simulink model "IEEE_BUS_68_AGC"  (R2025a)
settings: Solver=ode23tb  StartTime=0.0  StopTime=150  FixedStep=Ts  MaxStep=0.0001  RelTol=1e-3
PreLoadFcn:
  | PSSMODEL=1;
  | LPSS=0;
  | WAPSS=0;
  | WAPSS2=0;
  | Ts=50e-5;
InitFcn:
  | PSSMODEL=1;
  | LPSS=0;
  | WAPSS=0;
  | WAPSS2=0;
  | Ts=50e-5;
  | 
  | % Required data to 68 Bus benchmark
  | % clear
  | % clc
  | % Definition for the columns
  | % system base =100 MVA
  | 
  | %% Line data Format (line)
  | % All values are given on the same system base MVA
  | % 1: From bus
  | % 2: To bus
  | % 3: Resistance (pu)
  | % 4: Reactance  (pu)
  | % 5: Charge     (pu)
  | % 6: Transformer Tap Amplitute
  | % 7: base MVA
  | % 8: Nomonal Voltage (KV)
  | 
  | %1   2    3        4       5       6        7      8
  | line=[...
  | 1	54	0	     0.0181	  0	      1.025     100    13.8
  | 2	58	0	     0.025	  0	      1.070     100    13.8
  | 3	62	0	     0.02	  0	      1.070     100    13.8
  | 4	19	0.0007	 0.0142	  0	      1.070     100    13.8
  | 5	20	0.0009	 0.018	  0	      1.009     100    13.8
  | 6	22	0	     0.0143	  0	      1.025     100    13.8
  | 7	23	0.0005	 0.0272	  0	      0         100    13.8
  | 8	25	0.0006	 0.0232	  0	      1.025     100    13.8
  | 9	29	0.0008	 0.0156   0	      1.025     100    13.8
  | 10	31	0	     0.026	  0	      1.04      100    13.8
  | 11	32	0	     0.013	  0	      1.04      100    13.8
  | 12	36	0	     0.0075	  0	      1.04      100    13.8
  | 13	17	0	     0.0033	  0	      1.04      100    13.8
  | 14	41	0	     0.0015	  0	      1         100    13.8
  | 15	42	0	     0.0015	  0	      1         100    13.8
  | 16	18	0	     0.003	  0	      1         100    13.8
  | 17	36	0.0005	 0.0045	  0.32	  0         100    138
  | 17	43	0.0005	 0.0276	  0	      0         100    138
  | 18	42	0.004	 0.06	  2.25    0         100    138
  | 18	49	0.0076	 0.1141	  1.16    0	        100    138
  | 18	50	0.0012	 0.0288	  2.06	  0         100    138
  | 20	19	0.0007	 0.0138	  0       1.06	    100    138
  | 19	68	0.0016	 0.0195	  0.304	  0         100    138
  | 21	22	0.0008	 0.014	  0.2565  0	        100    138
  | 21	68	0.0008	 0.0135	  0.2548  0	        100    138
  | 22	23	0.0006	 0.0096	  0.1846  0	        100    138
  | 23	24	0.0022	 0.035	  0.361	  0         100    138
  | 24	68	0.0003	 0.0059	  0.068	  0         100    138
  | 25	26	0.0032	 0.0323	  0.531	  0         100    138
  | 25	54	0.007	 0.0086	  0.146	  0         100    138
  | 26	27	0.0014	 0.0147	  0.2396  0	        100    138
  | 26	28	0.0043	 0.0474	  0.7802  0	        100    138
  | 26	29	0.0057	 0.0625	  1.029	  0         100    138
  | 27	37	0.0013	 0.0173	  0.3216  0	        100    138
  | 27	53	0.032	 0.32	  0.41	  0         100    138
  | ... (+206 lines)
undefined symbols (not defined in the file or in its folder): D1, Delta
libraries: spsPMUPLLBasedPositiveSequenceLib x90, spsRMSLib x73, spsThreePhaseVIMeasurementLib x69, spsLoadFlowBusLib x69, spsThreePhasePISectionLineLib x64, spsThreePhaseParallelRLCLoadLib x35, spsGenericPowerSystemStabilizerLib x32, spsThreePhaseSeriesRLCLoadLib x21, spsThreePhaseTransformerTwoWindingsLib x21, spsSynchronousMachinepuStandardLib x20, spsExcitationSystemLib x16, spsMultiBandPowerSystemStabilizerLib x16
(part 2 of 8)

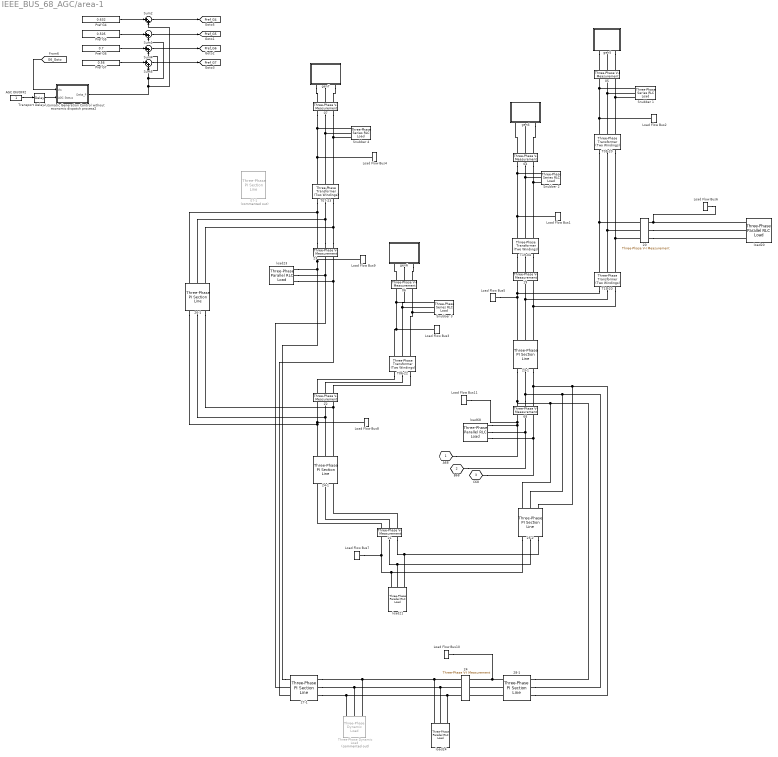
== system IEEE_BUS_68_AGC/area-1 ==
  04 : spsThreePhaseVIMeasurementLib/Three-Phase V-I Measurement  VoltageMeasurement=phase-to-phase  SetLabelV=on  LabelV=Vabc_04  Vpu=off  VpuLL=on  CurrentMeasurement=no  SetLabelI=off  LabelI=Iabc  Ipu=off  Pbase=100e6  Vbase=13.8*1e3  OutputType=Complex  PhasorSimulation=off  PSBequivalent=0
  05 : spsThreePhaseVIMeasurementLib/Three-Phase V-I Measurement  VoltageMeasurement=phase-to-phase  SetLabelV=on  LabelV=Vabc_05  Vpu=off  VpuLL=on  CurrentMeasurement=no  SetLabelI=off  LabelI=Iabc  Ipu=off  Pbase=100e6  Vbase=13.8e3  OutputType=Complex  PhasorSimulation=off  PSBequivalent=0
  06 : spsThreePhaseVIMeasurementLib/Three-Phase V-I Measurement  VoltageMeasurement=phase-to-phase  SetLabelV=on  LabelV=Vabc_06  Vpu=off  VpuLL=on  CurrentMeasurement=no  SetLabelI=off  LabelI=Iabc  Ipu=off  Pbase=100e6  Vbase=13.8e3  OutputType=Complex  PhasorSimulation=off  PSBequivalent=0
  07 : spsThreePhaseVIMeasurementLib/Three-Phase V-I Measurement  VoltageMeasurement=phase-to-phase  SetLabelV=on  LabelV=Vabc_07  Vpu=off  VpuLL=on  CurrentMeasurement=no  SetLabelI=off  LabelI=Iabc  Ipu=off  Pbase=100e6  Vbase=13.8e3  OutputType=Complex  PhasorSimulation=off  PSBequivalent=0
  07-1 : spsThreePhasePISectionLineLib/Three-Phase PI Section Line  Commented=on  LConnTagsString=a|b|c  RConnTagsString=A|B|C  Length=1  Frequency=60  Resistances=[line(7,3) 3*line(7,3)]  Inductances=[line(7,4) 3*line(7,4)]  Capacitances=[line(28,5) line(28,5)/3]
  19 : spsThreePhaseVIMeasurementLib/Three-Phase V-I Measurement  VoltageMeasurement=phase-to-phase  SetLabelV=on  LabelV=Vabc_19  Vpu=off  VpuLL=on  CurrentMeasurement=no  SetLabelI=off  LabelI=Iabc  Ipu=off  Pbase=100e6  Vbase=Bus(19,2)*1e3  OutputType=Complex  PhasorSimulation=off  PSBequivalent=0
  20 : spsThreePhaseVIMeasurementLib/Three-Phase V-I Measurement  VoltageMeasurement=phase-to-phase  SetLabelV=on  LabelV=Vabc_20  Vpu=off  VpuLL=on  CurrentMeasurement=no  SetLabelI=off  LabelI=Iabc  Ipu=off  Pbase=100e6  Vbase=Bus(20,2)*1e3  OutputType=Complex  PhasorSimulation=off  PSBequivalent=0
  21 : spsThreePhaseVIMeasurementLib/Three-Phase V-I Measurement  VoltageMeasurement=phase-to-phase  SetLabelV=on  LabelV=Vabc_21  Vpu=off  VpuLL=on  CurrentMeasurement=no  SetLabelI=off  LabelI=Iabc  Ipu=off  Pbase=100e6  Vbase=Bus(21,2)*1e3  OutputType=Complex  PhasorSimulation=off  PSBequivalent=0
  22 : spsThreePhaseVIMeasurementLib/Three-Phase V-I Measurement  VoltageMeasurement=phase-to-phase  SetLabelV=on  LabelV=Vabc_22  Vpu=off  VpuLL=on  CurrentMeasurement=no  SetLabelI=off  LabelI=Iabc  Ipu=off  Pbase=100e6  Vbase=Bus(22,2)*1e3  OutputType=Complex  PhasorSimulation=off  PSBequivalent=0
  23 : spsThreePhaseVIMeasurementLib/Three-Phase V-I Measurement  VoltageMeasurement=phase-to-phase  SetLabelV=on  LabelV=Vabc_23  Vpu=off  VpuLL=on  CurrentMeasurement=no  SetLabelI=off  LabelI=Iabc  Ipu=off  Pbase=100e6  Vbase=Bus(23,2)*1e3  OutputType=Complex  PhasorSimulation=off  PSBequivalent=0
  23-1 : spsThreePhasePISectionLineLib/Three-Phase PI Section Line  LConnTagsString=a|b|c  RConnTagsString=A|B|C  Length=1  Frequency=60  Resistances="[line(23,3)  3*line(23,3)]"  Inductances=[line(23,4) 3*line(23,4)]  Capacitances=[line(23,5) line(23,5)/3]
  24 : spsThreePhaseVIMeasurementLib/Three-Phase V-I Measurement  VoltageMeasurement=phase-to-phase  SetLabelV=on  LabelV=Vabc_24  Vpu=off  VpuLL=on  CurrentMeasurement=no  SetLabelI=off  LabelI=Iabc  Ipu=off  Pbase=100e6  Vbase=Bus(24,2)*1e3  OutputType=Complex  PhasorSimulation=off  PSBequivalent=0
  24-1 : spsThreePhasePISectionLineLib/Three-Phase PI Section Line  LConnTagsString=a|b|c  RConnTagsString=A|B|C  Length=1  Frequency=60  Resistances=[line(24,3) 3*line(24,3)]  Inductances=[line(24,4) 3*line(24,4)]  Capacitances=[line(24,5) line(24,5)/3]
  25-2 : spsThreePhasePISectionLineLib/Three-Phase PI Section Line  LConnTagsString=a|b|c  RConnTagsString=A|B|C  Length=1  Frequency=60  Resistances=[line(25,3) 3*line(25,3)]  Inductances=[line(25,4) 3*line(25,4)]  Capacitances=[line(25,5) line(25,5)/3]
  26-1 : spsThreePhasePISectionLineLib/Three-Phase PI Section Line  LConnTagsString=a|b|c  RConnTagsString=A|B|C  Length=1  Frequency=60  Resistances=[line(26,3) 3*line(26,3)]  Inductances=[line(26,4) 3*line(26,4)]  Capacitances=[line(26,5) line(26,5)/3]
  27-1 : spsThreePhasePISectionLineLib/Three-Phase PI Section Line  LConnTagsString=a|b|c  RConnTagsString=A|B|C  Length=1  Frequency=60  Resistances=[line(27,3) 3*line(27,3)]  Inductances=[line(27,4) 3*line(27,4)]  Capacitances=[line(27,5) line(27,5)/3]
  28-1 : spsThreePhasePISectionLineLib/Three-Phase PI Section Line  LConnTagsString=a|b|c  RConnTagsString=A|B|C  Length=1  Frequency=60  Resistances=[line(28,3) 3*line(28,3)]  Inductances=[line(28,4) 3*line(28,4)]  Capacitances=[line(28,5) line(28,5)/3]
  68 : spsThreePhaseVIMeasurementLib/Three-Phase V-I Measurement  VoltageMeasurement=phase-to-phase  SetLabelV=on  LabelV=Vabc_68  Vpu=off  VpuLL=on  CurrentMeasurement=no  SetLabelI=off  LabelI=Iabc  Ipu=off  Pbase=100e6  Vbase=Bus(68,2)*1e3  OutputType=Complex  PhasorSimulation=off  PSBequivalent=0
  AGC ON/OFF2 : Constant
  Automatic Generation Control without economic dispatch process2 : Subsystem
  Load Flow Bus1 : spsLoadFlowBusLib/Load Flow Bus  LConnTagsString=a  Phases=single  Connectors=on one side  ID=BUS_04  Vbase=13.8e3  Vref=0.997  Vangle=0  VLF=0.997  VLFb=1  VLFc=1  angleLF=-1.084  angleLFb=0  angleLFc=0
  Load Flow Bus10 : spsLoadFlowBusLib/Load Flow Bus  LConnTagsString=a  Phases=single  Connectors=on one side  ID=BUS_24  Vbase=138e3  Vref=1  Vangle=0  VLF=1.017  VLFb=1  VLFc=1  angleLF=18.89  angleLFb=0  angleLFc=0
  Load Flow Bus11 : spsLoadFlowBusLib/Load Flow Bus  LConnTagsString=a  Phases=single  Connectors=on one side  ID=BUS_68  Vbase=138e3  Vref=1  Vangle=0  VLF=1.009  VLFb=1  VLFc=1  angleLF=18.71  angleLFb=0  angleLFc=0
  Load Flow Bus2 : spsLoadFlowBusLib/Load Flow Bus  LConnTagsString=a  Phases=single  Connectors=on one side  ID=BUS_05  Vbase=13.8e3  Vref=1.011  Vangle=0  VLF=1.011  VLFb=1  VLFc=1  angleLF=-5.107  angleLFb=0  angleLFc=0
  Load Flow Bus3 : spsLoadFlowBusLib/Load Flow Bus  LConnTagsString=a  Phases=single  Connectors=on one side  ID=BUS_06  Vbase=13.8e3  Vref=1.05  Vangle=0  VLF=1.05  VLFb=1  VLFc=1  angleLF=-1.181  angleLFb=0  angleLFc=0
  Load Flow Bus4 : spsLoadFlowBusLib/Load Flow Bus  LConnTagsString=a  Phases=single  Connectors=on one side  ID=BUS_07  Vbase=13.8e3  Vref=1.063  Vangle=0  VLF=1.063  VLFb=1  VLFc=1  angleLF=-0.2085  angleLFb=0  angleLFc=0
  Load Flow Bus5 : spsLoadFlowBusLib/Load Flow Bus  LConnTagsString=a  Phases=single  Connectors=on one side  ID=BUS_19  Vbase=138e3  Vref=1  Vangle=0  VLF=0.9998  VLFb=1  VLFc=1  angleLF=23.76  angleLFb=0  angleLFc=0
  Load Flow Bus6 : spsLoadFlowBusLib/Load Flow Bus  LConnTagsString=a  Phases=single  Connectors=on one side  ID=BUS_20  Vbase=138e3  Vref=1  Vangle=0  VLF=0.9971  VLFb=1  VLFc=1  angleLF=22.34  angleLFb=0  angleLFc=0
  Load Flow Bus7 : spsLoadFlowBusLib/Load Flow Bus  LConnTagsString=a  Phases=single  Connectors=on one side  ID=BUS_21  Vbase=138e3  Vref=1  Vangle=0  VLF=1.014  VLFb=1  VLFc=1  angleLF=21.41  angleLFb=0  angleLFc=0
  Load Flow Bus8 : spsLoadFlowBusLib/Load Flow Bus  LConnTagsString=a  Phases=single  Connectors=on one side  ID=BUS_22  Vbase=138e3  Vref=1  Vangle=0  VLF=1.039  VLFb=1  VLFc=1  angleLF=26.18  angleLFb=0  angleLFc=0
  Load Flow Bus9 : spsLoadFlowBusLib/Load Flow Bus  LConnTagsString=a  Phases=single  Connectors=on one side  ID=BUS_23  Vbase=138e3  Vref=1  Vangle=0  VLF=1.039  VLFb=1  VLFc=1  angleLF=25.85  angleLFb=0  angleLFc=0
  Pref G4 : Constant  Value=0.632
  Pref G5 : Constant  Value=0.505
  Pref G6 : Constant  Value=0.7
  Pref G7 : Constant  Value=0.56
  Snubber {1..4} (4 alike) : spsThreePhaseSeriesRLCLoadLib/Three-Phase Series RLC Load  LConnTagsString=A|B|C  Configuration=Y (grounded)  NominalVoltage=13.8e3  Vabc=[1e3 1e3 1e3]  Vabcp=[1e3 1e3 1e3]  NominalFrequency=60  UnbalancedPower=off  ActivePower=1000000  InductivePower=0  CapacitivePower=10000000  Pabc=[10e3 9e3 11e3]  QLabc=[100 90 110]  QCabc=[100 90 110]  Pabcp=[10e3 9e3 11e3]  QLabcp=[100 90 110]  QCabcp=[100 90 110]  Measurements=None  LoadType=constant Z
  Sum{1..2,4..5} (4 alike) : Sum  Inputs=|++
  T05-20 : spsThreePhaseTransformerTwoWindingsLib/Three-Phase Transformer (Two Windings)  Winding1Connection=Delta (D1)  Winding2Connection=Yg  CoreType=Three single-phase transformers  SetSaturation=off  Hysteresis=off  DataFile='hysteresis'  SetInitialFlux=off  Measurements=None  UNITS=pu  NominalPower=[ 100e6 , 60 ]  Winding1=[ 13.8e3 , 0.0, 0 ]  Winding2=[ 138e3 , 0.00085, 0.0091]  Rm=500  Lm=500  L0=0.5  Saturation=[ 0,0 ; 0.0024,1.2 ; 1.0,1.52 ]  InitialFluxes=[ 0.8 , -0.8 , 0.7 ]  BreakLoop=off  DiscreteSolver=Trapezoidal robust  DataType=off  TransfoNumber=1
  T06-22 : spsThreePhaseTransformerTwoWindingsLib/Three-Phase Transformer (Two Windings)  Winding1Connection=Delta (D1)  Winding2Connection=Yg  CoreType=Three single-phase transformers  SetSaturation=off  Hysteresis=off  DataFile='hysteresis'  SetInitialFlux=off  Measurements=None  UNITS=pu  NominalPower=[ 100e6 , 60 ]  Winding1=[ 13.8e3 , 0.00 , 0 ]  Winding2=[ 138e3 , 0.000 , 0.0072 ]  Rm=500  Lm=500  L0=0.5  Saturation=[ 0,0 ; 0.0024,1.2 ; 1.0,1.52 ]  InitialFluxes=[ 0.8 , -0.8 , 0.7 ]  BreakLoop=off  DiscreteSolver=Trapezoidal robust  DataType=off  TransfoNumber=1
  T07-23 : spsThreePhaseTransformerTwoWindingsLib/Three-Phase Transformer (Two Windings)  Winding1Connection=Delta (D1)  Winding2Connection=Yg  CoreType=Three single-phase transformers  SetSaturation=off  Hysteresis=off  DataFile='hysteresis'  SetInitialFlux=off  Measurements=None  UNITS=pu  NominalPower=[ 100e6 , 60 ]  Winding1=[ 13.8e3 , 0.00035 , 0 ]  Winding2=[ 138e3 , 0.00035, 0.0138]  Rm=500  Lm=500  L0=0.5  Saturation=[ 0,0 ; 0.0024,1.2 ; 1.0,1.52 ]  InitialFluxes=[ 0.8 , -0.8 , 0.7 ]  BreakLoop=off  DiscreteSolver=Trapezoidal robust  DataType=off  TransfoNumber=1
  T19-04 : spsThreePhaseTransformerTwoWindingsLib/Three-Phase Transformer (Two Windings)  Winding1Connection=Delta (D1)  Winding2Connection=Yg  CoreType=Three single-phase transformers  SetSaturation=off  Hysteresis=off  DataFile='hysteresis'  SetInitialFlux=off  Measurements=None  UNITS=pu  NominalPower=[ 100e6 , 60 ]  Winding1=[ 13.8e3 , 0.00035 , 0 ]  Winding2=[ 138e3 , 0.000035, 0.0142]  Rm=500  Lm=500  L0=0.5  Saturation=[ 0,0 ; 0.0024,1.2 ; 1.0,1.52 ]  InitialFluxes=[ 0.8 , -0.8 , 0.7 ]  BreakLoop=off  DiscreteSolver=Trapezoidal robust  DataType=off  TransfoNumber=1
  T19-20 : spsThreePhaseTransformerTwoWindingsLib/Three-Phase Transformer (Two Windings)  Winding1Connection=Y  Winding2Connection=Y  CoreType=Three single-phase transformers  SetSaturation=off  Hysteresis=off  DataFile='hysteresis'  SetInitialFlux=off  Measurements=None  UNITS=pu  NominalPower=[ 100e6 , 60 ]  Winding1=[ 138e3 , 0.00035 , 0 ]  Winding2=[ 138e3 , 0.00035, 0.0138]  Rm=500  Lm=500  L0=0.5  Saturation=[ 0,0 ; 0.0024,1.2 ; 1.0,1.52 ]  InitialFluxes=[ 0.8 , -0.8 , 0.7 ]  BreakLoop=off  DiscreteSolver=Trapezoidal robust  DataType=off  TransfoNumber=1
  Three-Phase Dynamic Load : spsThreePhaseDynamicLoadLib/Three-Phase Dynamic Load  Commented=on  NominalVoltage=[138000 60 ]  ActiveReactivePowers=[309000000 -92000000]  PositiveSequence=[1.01116 21.5615]  ExternalControl=off  NpNq=[1.3 2]  TimeConstants=[0.1 0.1 0.1 0.1]  MinimumVoltage=0.5  Tfilter=0.01  LoadFlowParameters=[4,0,0,0,0]
      settings: LibrarySourceBlock=|
      | sps_lib/Passives/Three-Phase
      | Dynamic Load
  Transport Delay2 : TransportDelay  DelayTime=20
  gen4 : Subsystem
  gen5 : Subsystem
  gen6 : Subsystem
  gen7 : Subsystem
  load20 : spsThreePhaseParallelRLCLoadLib/Three-Phase Parallel RLC Load  LConnTagsString=A|B|C  Configuration=Y (grounded)  NominalVoltage=(138000)*0.997073  Vabc=[1e3 1e3 1e3]  Vabcp=[1e3 1e3 1e3]  NominalFrequency=60  UnbalancedPower=off  ActivePower=680000000  InductivePower=103000000  CapacitivePower=0  Pabc=[10e3 9e3 11e3]  QLabc=[100 90 110]  QCabc=[100 90 110]  Pabcp=[10e3 9e3 11e3]  QLabcp=[100 90 110]  QCabcp=[100 90 110]  Measurements=None  LoadType=constant PQ
  load21 : spsThreePhaseParallelRLCLoadLib/Three-Phase Parallel RLC Load  LConnTagsString=A|B|C  Configuration=Y (grounded)  NominalVoltage=(138000)*1.01427  Vabc=[1e3 1e3 1e3]  Vabcp=[1e3 1e3 1e3]  NominalFrequency=60  UnbalancedPower=off  ActivePower=274000000  InductivePower=115000000  CapacitivePower=0  Pabc=[10e3 9e3 11e3]  QLabc=[100 90 110]  QCabc=[100 90 110]  Pabcp=[10e3 9e3 11e3]  QLabcp=[100 90 110]  QCabcp=[100 90 110]  Measurements=None  LoadType=constant PQ
  load23 : spsThreePhaseParallelRLCLoadLib/Three-Phase Parallel RLC Load  LConnTagsString=A|B|C  Configuration=Y (grounded)  NominalVoltage=(138000)*1.03943  Vabc=[1e3 1e3 1e3]  Vabcp=[1e3 1e3 1e3]  NominalFrequency=60  UnbalancedPower=off  ActivePower=248000000  InductivePower=85000000  CapacitivePower=0  Pabc=[10e3 9e3 11e3]  QLabc=[100 90 110]  QCabc=[100 90 110]  Pabcp=[10e3 9e3 11e3]  QLabcp=[100 90 110]  QCabcp=[100 90 110]  Measurements=None  LoadType=constant PQ
  load24 : spsThreePhaseParallelRLCLoadLib/Three-Phase Parallel RLC Load  LConnTagsString=A|B|C  Configuration=Y (grounded)  NominalVoltage=(138000)*1.01674  Vabc=[1e3 1e3 1e3]  Vabcp=[1e3 1e3 1e3]  NominalFrequency=60  UnbalancedPower=off  ActivePower=309000000  InductivePower=0  CapacitivePower=92000000  Pabc=[10e3 9e3 11e3]  QLabc=[100 90 110]  QCabc=[100 90 110]  Pabcp=[10e3 9e3 11e3]  QLabcp=[100 90 110]  QCabcp=[100 90 110]  Measurements=None  LoadType=constant PQ
  load68 : spsThreePhaseParallelRLCLoadLib/Three-Phase Parallel RLC Load  LConnTagsString=A|B|C  Configuration=Y (grounded)  NominalVoltage=(138000)*1.00875  Vabc=[1e3 1e3 1e3]  Vabcp=[1e3 1e3 1e3]  NominalFrequency=60  UnbalancedPower=off  ActivePower=329000000  InductivePower=32000000  CapacitivePower=0  Pabc=[10e3 9e3 11e3]  QLabc=[100 90 110]  QCabc=[100 90 110]  Pabcp=[10e3 9e3 11e3]  QLabcp=[100 90 110]  QCabcp=[100 90 110]  Measurements=None  LoadType=constant PQ
  A68 : PMIOPort  Tag=PMCPort  Side=Right
  B68 : PMIOPort  Tag=PMCPort  Port=2  Side=Right
  C68 : PMIOPort  Tag=PMCPort  Port=3  Side=Right
  tag scope: Pref_G4=global, Pref_G5=global, Pref_G6=global, Pref_G7=global
  wires:
  Sum2/1 -> [Pref_G4]
  Sum1/1 -> [Pref_G5]
  Pref G6/1 -> Sum4/1
  Sum5/1 -> [Pref_G7]
  Automatic Generation Control without economic dispatch process2/1(Delta_P) -> Sum2/2, Sum1/2, Sum4/2, Sum5/2
  Pref G4/1 -> Sum2/1
  Sum4/1 -> [Pref_G6]
  Pref G5/1 -> Sum1/1
  Pref G7/1 -> Sum5/1
  [G6_Goto] -> Automatic Generation Control without economic dispatch process2/1(dw)
  AGC ON/OFF2/1 -> Transport Delay2/1
  Transport Delay2/1 -> Automatic Generation Control without economic dispatch process2/2(AGC Status)
  ? -> ?
  ? -> ?
  ? -> ?
  ? -> ?
  connections:
  B68/RConn1 -- load68/LConn2 -- 68/LConn2
  27-1/LConn1 -- Load Flow Bus9/LConn1 -- 23/LConn1 -- load23/LConn1
  T19-20/LConn3 -- T05-20/RConn3 -- 20/RConn3
  20/RConn1 -- T05-20/RConn1 -- T19-20/LConn1
  24-1/RConn1 -- 26-1/RConn1 -- Load Flow Bus8/LConn1 -- 22/LConn1
  04/LConn2 -- T19-04/LConn2 -- Snubber 2/LConn2
  07/LConn1 -- Snubber 4/LConn1 -- Load Flow Bus4/LConn1 -- T07-23/LConn1
  07/LConn3 -- T07-23/LConn3 -- Snubber 4/LConn3
  load23/LConn2 -- 23/LConn2 -- 27-1/LConn2
  21/LConn3 -- load21/LConn3 -- 25-2/RConn3
  24-1/RConn3 -- 22/LConn3 -- 26-1/RConn3
  04/LConn1 -- Snubber 2/LConn1 -- Load Flow Bus1/LConn1 -- T19-04/LConn1
  A68/RConn1 -- load68/LConn1 -- 68/LConn1 -- Load Flow Bus11/LConn1
  04/RConn1 -- gen4/LConn1
  T19-20/LConn2 -- T05-20/RConn2 -- 20/RConn2
  23-1/RConn1 -- Load Flow Bus5/LConn1 -- T19-20/RConn1 -- 19/LConn1
  21/LConn2 -- load21/LConn2 -- 25-2/RConn2
  load23/LConn3 -- 23/LConn3 -- 27-1/LConn3
  T06-22/RConn3 -- 22/RConn3
  07/LConn2 -- Snubber 4/LConn2 -- T07-23/LConn2
  load21/LConn1 -- Load Flow Bus7/LConn1 -- 21/LConn1 -- 25-2/RConn1
  C68/RConn1 -- load68/LConn3 -- 68/LConn3
  T06-22/LConn1 -- Load Flow Bus3/LConn1 -- Snubber 3/LConn1 -- 06/LConn1
  T05-20/LConn1 -- Load Flow Bus2/LConn1 -- Snubber 1/LConn1 -- 05/LConn1
  T06-22/LConn3 -- 06/LConn3 -- Snubber 3/LConn3
  26-1/RConn2 -- 24-1/RConn2 -- 22/LConn2
  T06-22/LConn2 -- Snubber 3/LConn2 -- 06/LConn2
  04/LConn3 -- Snubber 2/LConn3 -- T19-04/LConn3
  T06-22/RConn2 -- 22/RConn2
  gen4/LConn2 -- 04/RConn2
  23-1/LConn1 -- 68/RConn1 -- 28-1/LConn1 -- 25-2/LConn1
  T19-04/RConn3 -- 19/RConn3
  68/RConn2 -- 23-1/LConn2 -- 28-1/LConn2 -- 25-2/LConn2
  T06-22/RConn1 -- 22/RConn1
  T19-04/RConn2 -- 19/RConn2
  28-1/LConn3 -- 68/RConn3 -- 23-1/LConn3 -- 25-2/LConn3
  gen4/LConn3 -- 04/RConn3
  19/LConn2 -- 23-1/RConn2 -- T19-20/RConn2
  T19-04/RConn1 -- 19/RConn1
  T05-20/LConn2 -- Snubber 1/LConn2 -- 05/LConn2
  T05-20/LConn3 -- Snubber 1/LConn3 -- 05/LConn3
  gen5/LConn1 -- 05/RConn1
  gen5/LConn2 -- 05/RConn2
  gen5/LConn3 -- 05/RConn3
  06/RConn1 -- gen6/LConn1
  gen6/LConn2 -- 06/RConn2
  gen6/LConn3 -- 06/RConn3
  gen7/LConn1 -- 07/RConn1
  gen7/LConn2 -- 07/RConn2
  gen7/LConn3 -- 07/RConn3
  19/LConn3 -- 23-1/RConn3 -- T19-20/RConn3
  23/RConn1 -- T07-23/RConn1 -- 26-1/LConn1
  23/RConn2 -- T07-23/RConn2 -- 26-1/LConn2
  23/RConn3 -- T07-23/RConn3 -- 26-1/LConn3
  21/RConn1 -- 24-1/LConn1
  21/RConn2 -- 24-1/LConn2
  21/RConn3 -- 24-1/LConn3
  28-1/RConn1 -- 24/LConn1 -- Load Flow Bus10/LConn1
  28-1/RConn2 -- 24/LConn2
  28-1/RConn3 -- 24/LConn3
  Load Flow Bus6/LConn1 -- load20/LConn1 -- 20/LConn1
  27-1/RConn1 -- load24/LConn1 -- 24/RConn1 -- Three-Phase Dynamic Load/LConn1
  24/RConn2 -- Three-Phase Dynamic Load/LConn2 -- 27-1/RConn2 -- load24/LConn2
  24/RConn3 -- Three-Phase Dynamic Load/LConn3 -- 27-1/RConn3 -- load24/LConn3
  20/LConn2 -- load20/LConn2
  20/LConn3 -- load20/LConn3

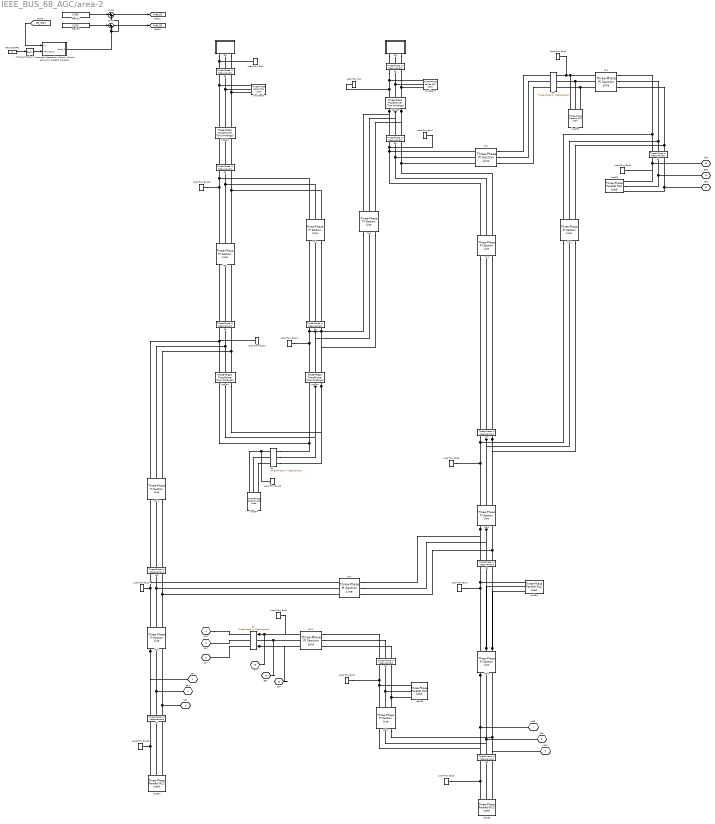
== system IEEE_BUS_68_AGC/area-2 ==
  02 : spsThreePhaseVIMeasurementLib/Three-Phase V-I Measurement  VoltageMeasurement=phase-to-phase  SetLabelV=on  LabelV=Vabc_02  Vpu=off  VpuLL=on  CurrentMeasurement=no  SetLabelI=off  LabelI=Iabc  Ipu=off  Pbase=100e6  Vbase=13.8e3  OutputType=Complex  PhasorSimulation=off  PSBequivalent=0
  03 : spsThreePhaseVIMeasurementLib/Three-Phase V-I Measurement  VoltageMeasurement=phase-to-phase  SetLabelV=on  LabelV=Vabc_03  Vpu=off  VpuLL=on  CurrentMeasurement=no  SetLabelI=off  LabelI=Iabc  Ipu=off  Pbase=100e6  Vbase=13.8e3  OutputType=Complex  PhasorSimulation=off  PSBequivalent=0
  37 : spsThreePhaseVIMeasurementLib/Three-Phase V-I Measurement  VoltageMeasurement=phase-to-phase  SetLabelV=on  LabelV=Vabc_37  Vpu=off  VpuLL=on  CurrentMeasurement=no  SetLabelI=off  LabelI=Iabc  Ipu=off  Pbase=100e6  Vbase=Bus(37,2)*1e3  OutputType=Complex  PhasorSimulation=off  PSBequivalent=0
  50-1 : spsThreePhasePISectionLineLib/Three-Phase PI Section Line  LConnTagsString=a|b|c  RConnTagsString=A|B|C  Length=1  Frequency=60  Resistances=[line(50,3) 3*line(50,3)]  Inductances=[line(50,4) 3*line(50,4)]  Capacitances=[line(50,5) line(50,5)/3]
  52 : spsThreePhaseVIMeasurementLib/Three-Phase V-I Measurement  VoltageMeasurement=phase-to-phase  SetLabelV=on  LabelV=Vabc_52  Vpu=off  VpuLL=on  CurrentMeasurement=no  SetLabelI=off  LabelI=Iabc  Ipu=off  Pbase=100e6  Vbase=Bus(52,2)*1e3  OutputType=Complex  PhasorSimulation=off  PSBequivalent=0
  55 : spsThreePhaseVIMeasurementLib/Three-Phase V-I Measurement  VoltageMeasurement=phase-to-phase  SetLabelV=on  LabelV=Vabc_55  Vpu=off  VpuLL=on  CurrentMeasurement=no  SetLabelI=off  LabelI=Iabc  Ipu=off  Pbase=100e6  Vbase=Bus(55,2)*1e3  OutputType=Complex  PhasorSimulation=off  PSBequivalent=0
  56 : spsThreePhaseVIMeasurementLib/Three-Phase V-I Measurement  VoltageMeasurement=phase-to-phase  SetLabelV=on  LabelV=Vabc_56  Vpu=off  VpuLL=on  CurrentMeasurement=no  SetLabelI=off  LabelI=Iabc  Ipu=off  Pbase=100e6  Vbase=Bus(56,2)*1e3  OutputType=Complex  PhasorSimulation=off  PSBequivalent=0
  57 : spsThreePhaseVIMeasurementLib/Three-Phase V-I Measurement  VoltageMeasurement=phase-to-phase  SetLabelV=on  LabelV=Vabc_57  Vpu=off  VpuLL=on  CurrentMeasurement=no  SetLabelI=off  LabelI=Iabc  Ipu=off  Pbase=100e6  Vbase=Bus(57,2)*1e3  OutputType=Complex  PhasorSimulation=off  PSBequivalent=0
  58 : spsThreePhaseVIMeasurementLib/Three-Phase V-I Measurement  VoltageMeasurement=phase-to-phase  SetLabelV=on  LabelV=Vabc_58  Vpu=off  VpuLL=on  CurrentMeasurement=no  SetLabelI=off  LabelI=Iabc  Ipu=off  Pbase=100e6  Vbase=Bus(58,2)*1e3  OutputType=Complex  PhasorSimulation=off  PSBequivalent=0
  59 : spsThreePhaseVIMeasurementLib/Three-Phase V-I Measurement  VoltageMeasurement=phase-to-phase  SetLabelV=on  LabelV=Vabc_59  Vpu=off  VpuLL=on  CurrentMeasurement=no  SetLabelI=off  LabelI=Iabc  Ipu=off  Pbase=100e6  Vbase=Bus(59,2)*1e3  OutputType=Complex  PhasorSimulation=off  PSBequivalent=0
  60 : spsThreePhaseVIMeasurementLib/Three-Phase V-I Measurement  VoltageMeasurement=phase-to-phase  SetLabelV=on  LabelV=Vabc_60  Vpu=off  VpuLL=on  CurrentMeasurement=no  SetLabelI=off  LabelI=Iabc  Ipu=off  Pbase=100e6  Vbase=Bus(60,2)*1e3  OutputType=Complex  PhasorSimulation=off  PSBequivalent=0
  62 : spsThreePhaseVIMeasurementLib/Three-Phase V-I Measurement  VoltageMeasurement=phase-to-phase  SetLabelV=on  LabelV=Vabc_62  Vpu=off  VpuLL=on  CurrentMeasurement=no  SetLabelI=off  LabelI=Iabc  Ipu=off  Pbase=100e6  Vbase=Bus(62,2)*1e3  OutputType=Complex  PhasorSimulation=off  PSBequivalent=0
  63 : spsThreePhaseVIMeasurementLib/Three-Phase V-I Measurement  VoltageMeasurement=phase-to-phase  SetLabelV=on  LabelV=Vabc_63  Vpu=off  VpuLL=on  CurrentMeasurement=no  SetLabelI=off  LabelI=Iabc  Ipu=off  Pbase=100e6  Vbase=Bus(63,2)*1e3  OutputType=Complex  PhasorSimulation=off  PSBequivalent=0
  64 : spsThreePhaseVIMeasurementLib/Three-Phase V-I Measurement  VoltageMeasurement=phase-to-phase  SetLabelV=on  LabelV=Vabc_64  Vpu=off  VpuLL=on  CurrentMeasurement=no  SetLabelI=off  LabelI=Iabc  Ipu=off  Pbase=100e6  Vbase=Bus(64,2)*1e3  OutputType=Complex  PhasorSimulation=off  PSBequivalent=0
  65 : spsThreePhaseVIMeasurementLib/Three-Phase V-I Measurement  VoltageMeasurement=phase-to-phase  SetLabelV=on  LabelV=Vabc_65  Vpu=off  VpuLL=on  CurrentMeasurement=no  SetLabelI=off  LabelI=Iabc  Ipu=off  Pbase=100e6  Vbase=Bus(65,2)*1e3  OutputType=Complex  PhasorSimulation=off  PSBequivalent=0
  65-1 : spsThreePhasePISectionLineLib/Three-Phase PI Section Line  LConnTagsString=a|b|c  RConnTagsString=A|B|C  Length=1  Frequency=60  Resistances=[line(65,3) 3*line(65,3)]  Inductances=[line(65,4) 3*line(65,4)]  Capacitances=[line(65,5) line(65,5)/3]
  66 : spsThreePhaseVIMeasurementLib/Three-Phase V-I Measurement  VoltageMeasurement=phase-to-phase  SetLabelV=on  LabelV=Vabc_66  Vpu=off  VpuLL=on  CurrentMeasurement=no  SetLabelI=off  LabelI=Iabc  Ipu=off  Pbase=100e6  Vbase=Bus(66,2)*1e3  OutputType=Complex  PhasorSimulation=off  PSBequivalent=0
  67 : spsThreePhaseVIMeasurementLib/Three-Phase V-I Measurement  VoltageMeasurement=phase-to-phase  SetLabelV=on  LabelV=Vabc_67  Vpu=off  VpuLL=on  CurrentMeasurement=no  SetLabelI=off  LabelI=Iabc  Ipu=off  Pbase=100e6  Vbase=Bus(67,2)*1e3  OutputType=Complex  PhasorSimulation=off  PSBequivalent=0
  68-1 : spsThreePhasePISectionLineLib/Three-Phase PI Section Line  LConnTagsString=a|b|c  RConnTagsString=A|B|C  Length=1  Frequency=60  Resistances=[line(68,3) 3*line(68,3)]  Inductances=[line(68,4) 3*line(68,4)]  Capacitances=[line(68,5) line(68,5)/3]
  69-1 : spsThreePhasePISectionLineLib/Three-Phase PI Section Line  LConnTagsString=a|b|c  RConnTagsString=A|B|C  Length=1  Frequency=60  Resistances=[line(69,3) 3*line(69,3)]  Inductances=[line(69,4) 3*line(69,4)]  Capacitances=[line(69,5) line(69,5)/3]
  70-1 : spsThreePhasePISectionLineLib/Three-Phase PI Section Line  LConnTagsString=a|b|c  RConnTagsString=A|B|C  Length=1  Frequency=60  Resistances=[line(70,3) 3*line(70,3)]  Inductances=[line(70,4) 3*line(70,4)]  Capacitances=[line(70,5) line(70,5)/3]
  71-1 : spsThreePhasePISectionLineLib/Three-Phase PI Section Line  LConnTagsString=a|b|c  RConnTagsString=A|B|C  Length=1  Frequency=60  Resistances=[line(71,3) 3*line(71,3)]  Inductances=[line(71,4) 3*line(71,4)]  Capacitances=[line(71,5) line(71,5)/3]
  72-1 : spsThreePhasePISectionLineLib/Three-Phase PI Section Line  LConnTagsString=a|b|c  RConnTagsString=A|B|C  Length=1  Frequency=60  Resistances=[line(72,3) 3*line(72,3)]  Inductances=[line(72,4) 3*line(72,4)]  Capacitances=[line(72,5) line(72,5)/3]
  73-1 : spsThreePhasePISectionLineLib/Three-Phase PI Section Line  LConnTagsString=a|b|c  RConnTagsString=A|B|C  Length=1  Frequency=60  Resistances=[line(73,3) 3*line(73,3)]  Inductances=[line(73,4) 3*line(73,4)]  Capacitances=[line(73,5) line(73,5)/3]
  74-1 : spsThreePhasePISectionLineLib/Three-Phase PI Section Line  LConnTagsString=a|b|c  RConnTagsString=A|B|C  Length=1  Frequency=60  Resistances=[line(74,3) 3*line(74,3)]  Inductances=[line(74,4) 3*line(74,4)]  Capacitances=[line(74,5) line(74,5)/3]
  75-1 : spsThreePhasePISectionLineLib/Three-Phase PI Section Line  LConnTagsString=a|b|c  RConnTagsString=A|B|C  Length=1  Frequency=60  Resistances=[line(75,3) 3*line(75,3)]  Inductances=[line(75,4) 3*line(75,4)]  Capacitances=[line(75,5) line(75,5)/3]
  77-1 : spsThreePhasePISectionLineLib/Three-Phase PI Section Line  LConnTagsString=a|b|c  RConnTagsString=A|B|C  Length=1  Frequency=60  Resistances=[line(77,3) 3*line(77,3)]  Inductances=[line(77,4) 3*line(77,4)]  Capacitances=[line(77,5) line(77,5)/3]
  78-1 : spsThreePhasePISectionLineLib/Three-Phase PI Section Line  LConnTagsString=a|b|c  RConnTagsString=A|B|C  Length=1  Frequency=60  Resistances=[line(78,3) 3*line(78,3)]  Inductances=[line(78,4) 3*line(78,4)]  Capacitances=[line(78,5) line(78,5)/3]
  81-1 : spsThreePhasePISectionLineLib/Three-Phase PI Section Line  LConnTagsString=a|b|c  RConnTagsString=A|B|C  Length=1  Frequency=60  Resistances=[line(81,3) 3*line(81,3)]  Inductances=[line(81,4) 3*line(81,4)]  Capacitances=[line(81,5) line(81,5)/3]
  81-2 : spsThreePhasePISectionLineLib/Three-Phase PI Section Line  LConnTagsString=a|b|c  RConnTagsString=A|B|C  Length=1  Frequency=60  Resistances=[line(81,3) 3*line(81,3)]  Inductances=[line(81,4) 3*line(81,4)]  Capacitances=[line(81,5) line(81,5)/3]
  AGC ON/OFF2 : Constant
  Automatic Generation Control without economic dispatch process2 : Subsystem
  G2 : Subsystem
  G3 : Subsystem
  Load Flow Bus : spsLoadFlowBusLib/Load Flow Bus  LConnTagsString=a  Phases=single  Connectors=on one side  ID=BUS_02  Vbase=13.8e3  Vref=0.98  Vangle=0  VLF=0.98  VLFb=1  VLFc=1  angleLF=-12.66  angleLFb=0  angleLFc=0
  Load Flow Bus1 : spsLoadFlowBusLib/Load Flow Bus  LConnTagsString=a  Phases=single  Connectors=on one side  ID=BUS_03  Vbase=13.8e3  Vref=0.983  Vangle=0  VLF=0.983  VLFb=1  VLFc=1  angleLF=-5.973  angleLFb=0  angleLFc=0
  Load Flow Bus10 : spsLoadFlowBusLib/Load Flow Bus  LConnTagsString=a  Phases=single  Connectors=on one side  ID=BUS_62  Vbase=138e3  Vref=1  Vangle=0  VLF=0.9822  VLFb=1  VLFc=1  angleLF=20.14  angleLFb=0  angleLFc=0
  Load Flow Bus11 : spsLoadFlowBusLib/Load Flow Bus  LConnTagsString=a  Phases=single  Connectors=on one side  ID=BUS_63  Vbase=138e3  Vref=1  Vangle=0  VLF=0.9798  VLFb=1  VLFc=1  angleLF=19.17  angleLFb=0  angleLFc=0
  Load Flow Bus12 : spsLoadFlowBusLib/Load Flow Bus  LConnTagsString=a  Phases=single  Connectors=on one side  ID=BUS_64  Vbase=138e3  Vref=1  Vangle=0  VLF=0.9711  VLFb=1  VLFc=1  angleLF=19.33  angleLFb=0  angleLFc=0
  Load Flow Bus13 : spsLoadFlowBusLib/Load Flow Bus  LConnTagsString=a  Phases=single  Connectors=on one side  ID=BUS_65  Vbase=138e3  Vref=1  Vangle=0  VLF=0.9826  VLFb=1  VLFc=1  angleLF=19.44  angleLFb=0  angleLFc=0
  Load Flow Bus14 : spsLoadFlowBusLib/Load Flow Bus  LConnTagsString=a  Phases=single  Connectors=on one side  ID=BUS_66  Vbase=138e3  Vref=1  Vangle=0  VLF=0.988  VLFb=1  VLFc=1  angleLF=17.89  angleLFb=0  angleLFc=0
  Load Flow Bus15 : spsLoadFlowBusLib/Load Flow Bus  LConnTagsString=a  Phases=single  Connectors=on one side  ID=BUS_67  Vbase=138e3  Vref=1  Vangle=0  VLF=0.9976  VLFb=1  VLFc=1  angleLF=17.99  angleLFb=0  angleLFc=0
  Load Flow Bus2 : spsLoadFlowBusLib/Load Flow Bus  LConnTagsString=a  Phases=single  Connectors=on one side  ID=BUS_52  Vbase=138e3  Vref=1  Vangle=0  VLF=1.005  VLFb=1  VLFc=1  angleLF=15.5  angleLFb=0  angleLFc=0
  Load Flow Bus3 : spsLoadFlowBusLib/Load Flow Bus  LConnTagsString=a  Phases=single  Connectors=on one side  ID=BUS_55  Vbase=138e3  Vref=1  Vangle=0  VLF=0.9931  VLFb=1  VLFc=1  angleLF=13.46  angleLFb=0  angleLFc=0
  Load Flow Bus4 : spsLoadFlowBusLib/Load Flow Bus  LConnTagsString=a  Phases=single  Connectors=on one side  ID=BUS_56  Vbase=138e3  Vref=1  Vangle=0  VLF=0.9815  VLFb=1  VLFc=1  angleLF=15.77  angleLFb=0  angleLFc=0
  Load Flow Bus5 : spsLoadFlowBusLib/Load Flow Bus  LConnTagsString=a  Phases=single  Connectors=on one side  ID=BUS_37  Vbase=138e3  Vref=1  Vangle=0  VLF=1.011  VLFb=1  VLFc=1  angleLF=16.75  angleLFb=0  angleLFc=0
  Load Flow Bus6 : spsLoadFlowBusLib/Load Flow Bus  LConnTagsString=a  Phases=single  Connectors=on one side  ID=BUS_57  Vbase=138e3  Vref=1  Vangle=0  VLF=0.9777  VLFb=1  VLFc=1  angleLF=16.56  angleLFb=0  angleLFc=0
  Load Flow Bus7 : spsLoadFlowBusLib/Load Flow Bus  LConnTagsString=a  Phases=single  Connectors=on one side  ID=BUS_58  Vbase=138e3  Vref=1  Vangle=0  VLF=0.9787  VLFb=1  VLFc=1  angleLF=17.29  angleLFb=0  angleLFc=0
  Load Flow Bus8 : spsLoadFlowBusLib/Load Flow Bus  LConnTagsString=a  Phases=single  Connectors=on one side  ID=BUS_59  Vbase=138e3  Vref=1  Vangle=0  VLF=0.9696  VLFb=1  VLFc=1  angleLF=14.76  angleLFb=0  angleLFc=0
  Load Flow Bus9 : spsLoadFlowBusLib/Load Flow Bus  LConnTagsString=a  Phases=single  Connectors=on one side  ID=BUS_60  Vbase=138e3  Vref=1  Vangle=0  VLF=0.9697  VLFb=1  VLFc=1  angleLF=14.12  angleLFb=0  angleLFc=0
  Pref G2 : Constant  Value=0.545
  Pref G3 : Constant  Value=0.325
  Snubber 8 : spsThreePhaseSeriesRLCLoadLib/Three-Phase Series RLC Load  LConnTagsString=A|B|C  Configuration=Y (grounded)  NominalVoltage=13.8e3  Vabc=[1e3 1e3 1e3]  Vabcp=[1e3 1e3 1e3]  NominalFrequency=60  UnbalancedPower=off  ActivePower=1000000  InductivePower=0  CapacitivePower=10000000  Pabc=[10e3 9e3 11e3]  QLabc=[100 90 110]  QCabc=[100 90 110]  Pabcp=[10e3 9e3 11e3]  QLabcp=[100 90 110]  QCabcp=[100 90 110]  Measurements=None  LoadType=constant Z
  Snubber 9 : spsThreePhaseSeriesRLCLoadLib/Three-Phase Series RLC Load  LConnTagsString=A|B|C  Configuration=Y (grounded)  NominalVoltage=13.8e3  Vabc=[1e3 1e3 1e3]  Vabcp=[1e3 1e3 1e3]  NominalFrequency=60  UnbalancedPower=off  ActivePower=1000000  InductivePower=0  CapacitivePower=10000000  Pabc=[10e3 9e3 11e3]  QLabc=[100 90 110]  QCabc=[100 90 110]  Pabcp=[10e3 9e3 11e3]  QLabcp=[100 90 110]  QCabcp=[100 90 110]  Measurements=None  LoadType=constant Z
  Sum4 : Sum  Inputs=|++
  Sum5 : Sum  Inputs=|++
  T02-58 : spsThreePhaseTransformerTwoWindingsLib/Three-Phase Transformer (Two Windings)  Winding1Connection=Delta (D1)  Winding2Connection=Yg  CoreType=Three single-phase transformers  SetSaturation=off  Hysteresis=off  DataFile='hysteresis'  SetInitialFlux=off  Measurements=None  UNITS=pu  NominalPower=[ 100e6 , 60 ]  Winding1=[ 13.8e3 , 0.0002 , 0 ]  Winding2=[ 138e3 , 0 .0002, 0.0125]  Rm=500  Lm=500  L0=0.5  Saturation=[ 0,0 ; 0.0024,1.2 ; 1.0,1.52 ]  InitialFluxes=[ 0.8 , -0.8 , 0.7 ]  BreakLoop=off  DiscreteSolver=Trapezoidal robust  DataType=off  TransfoNumber=1
  T03-62 : spsThreePhaseTransformerTwoWindingsLib/Three-Phase Transformer (Two Windings)  Winding1Connection=Delta (D1)  Winding2Connection=Yg  CoreType=Three single-phase transformers  SetSaturation=off  Hysteresis=off  DataFile='hysteresis'  SetInitialFlux=off  Measurements=None  UNITS=pu  NominalPower=[ 100e6 , 60 ]  Winding1=[ 13.8e3 , 0.000 , 0 ]  Winding2=[ 138e3 , 0.000, 0.0101]  Rm=500  Lm=500  L0=0.5  Saturation=[ 0,0 ; 0.0024,1.2 ; 1.0,1.52 ]  InitialFluxes=[ 0.8 , -0.8 , 0.7 ]  BreakLoop=off  DiscreteSolver=Trapezoidal robust  DataType=off  TransfoNumber=1
  T63-64 : spsThreePhaseTransformerTwoWindingsLib/Three-Phase Transformer (Two Windings)  Winding1Connection=Y  Winding2Connection=Y  CoreType=Three single-phase transformers  SetSaturation=off  Hysteresis=off  DataFile='hysteresis'  SetInitialFlux=off  Measurements=None  UNITS=pu  NominalPower=[ 100e6 , 60 ]  Winding1=[ 138e3 , 0.00152, 0 ]  Winding2=[ 138e3 , 0.00152 , 0.022]  Rm=500  Lm=500  L0=0.5  Saturation=[ 0,0 ; 0.0024,1.2 ; 1.0,1.52 ]  InitialFluxes=[ 0.8 , -0.8 , 0.7 ]  BreakLoop=off  DiscreteSolver=Trapezoidal robust  DataType=off  TransfoNumber=1
  T65-64 : spsThreePhaseTransformerTwoWindingsLib/Three-Phase Transformer (Two Windings)  Winding1Connection=Y  Winding2Connection=Y  CoreType=Three single-phase transformers  SetSaturation=off  Hysteresis=off  DataFile='hysteresis'  SetInitialFlux=off  Measurements=None  UNITS=pu  NominalPower=[ 100e6 , 60 ]  Winding1=[ 138e3 , 0.00152, 0 ]  Winding2=[ 138e3 , 0.00152 , 0.022]  Rm=500  Lm=500  L0=0.5  Saturation=[ 0,0 ; 0.0024,1.2 ; 1.0,1.52 ]  InitialFluxes=[ 0.8 , -0.8 , 0.7 ]  BreakLoop=off  DiscreteSolver=Trapezoidal robust  DataType=off  TransfoNumber=1
  Transport Delay2 : TransportDelay  DelayTime=20
  load52 : spsThreePhaseParallelRLCLoadLib/Three-Phase Parallel RLC Load  LConnTagsString=A|B|C  Configuration=Y (grounded)  NominalVoltage=(138000)*1.00456  Vabc=[1e3 1e3 1e3]  Vabcp=[1e3 1e3 1e3]  NominalFrequency=60  UnbalancedPower=off  ActivePower=2000000  InductivePower=460000  CapacitivePower=0  Pabc=[10e3 9e3 11e3]  QLabc=[100 90 110]  QCabc=[100 90 110]  Pabcp=[10e3 9e3 11e3]  QLabcp=[100 90 110]  QCabcp=[100 90 110]  Measurements=None  LoadType=constant PQ
  load55 : spsThreePhaseParallelRLCLoadLib/Three-Phase Parallel RLC Load  LConnTagsString=A|B|C  Configuration=Y (grounded)  NominalVoltage=(138000)*0.993139  Vabc=[1e3 1e3 1e3]  Vabcp=[1e3 1e3 1e3]  NominalFrequency=60  UnbalancedPower=off  ActivePower=680000000  InductivePower=157000000  CapacitivePower=0  Pabc=[10e3 9e3 11e3]  QLabc=[100 90 110]  QCabc=[100 90 110]  Pabcp=[10e3 9e3 11e3]  QLabcp=[100 90 110]  QCabcp=[100 90 110]  Measurements=None  LoadType=constant PQ
  load56 : spsThreePhaseParallelRLCLoadLib/Three-Phase Parallel RLC Load  LConnTagsString=A|B|C  Configuration=Y (grounded)  NominalVoltage=(138000)*0.981548  Vabc=[1e3 1e3 1e3]  Vabcp=[1e3 1e3 1e3]  NominalFrequency=60  UnbalancedPower=off  ActivePower=200000000  InductivePower=74000000  CapacitivePower=0  Pabc=[10e3 9e3 11e3]  QLabc=[100 90 110]  QCabc=[100 90 110]  Pabcp=[10e3 9e3 11e3]  QLabcp=[100 90 110]  QCabcp=[100 90 110]  Measurements=None  LoadType=constant PQ
  load59 : spsThreePhaseParallelRLCLoadLib/Three-Phase Parallel RLC Load  LConnTagsString=A|B|C  Configuration=Y (grounded)  NominalVoltage=(138000)*0.969624  Vabc=[1e3 1e3 1e3]  Vabcp=[1e3 1e3 1e3]  NominalFrequency=60  UnbalancedPower=off  ActivePower=234000000  InductivePower=84000000  CapacitivePower=0  Pabc=[10e3 9e3 11e3]  QLabc=[100 90 110]  QCabc=[100 90 110]  Pabcp=[10e3 9e3 11e3]  QLabcp=[100 90 110]  QCabcp=[100 90 110]  Measurements=None  LoadType=constant PQ
  load60 : spsThreePhaseParallelRLCLoadLib/Three-Phase Parallel RLC Load  LConnTagsString=A|B|C  Configuration=Y (grounded)  NominalVoltage=(138000)*0.969673  Vabc=[1e3 1e3 1e3]  Vabcp=[1e3 1e3 1e3]  NominalFrequency=60  UnbalancedPower=off  ActivePower=209000000  InductivePower=71000000  CapacitivePower=0  Pabc=[10e3 9e3 11e3]  QLabc=[100 90 110]  QCabc=[100 90 110]  Pabcp=[10e3 9e3 11e3]  QLabcp=[100 90 110]  QCabcp=[100 90 110]  Measurements=None  LoadType=constant PQ
  load64 : spsThreePhaseParallelRLCLoadLib/Three-Phase Parallel RLC Load  LConnTagsString=A|B|C  Configuration=Y (grounded)  NominalVoltage=(138000)*0.971077  Vabc=[1e3 1e3 1e3]  Vabcp=[1e3 1e3 1e3]  NominalFrequency=60  UnbalancedPower=off  ActivePower=9000000  InductivePower=88000000  CapacitivePower=0  Pabc=[10e3 9e3 11e3]  QLabc=[100 90 110]  QCabc=[100 90 110]  Pabcp=[10e3 9e3 11e3]  QLabcp=[100 90 110]  QCabcp=[100 90 110]  Measurements=None  LoadType=constant PQ
  load67 : spsThreePhaseParallelRLCLoadLib/Three-Phase Parallel RLC Load  LConnTagsString=A|B|C  Configuration=Y (grounded)  NominalVoltage=(138000)*0.997643  Vabc=[1e3 1e3 1e3]  Vabcp=[1e3 1e3 1e3]  NominalFrequency=60  UnbalancedPower=off  ActivePower=118000000  InductivePower=27000000  CapacitivePower=0  Pabc=[10e3 9e3 11e3]  QLabc=[100 90 110]  QCabc=[100 90 110]  Pabcp=[10e3 9e3 11e3]  QLabcp=[100 90 110]  QCabcp=[100 90 110]  Measurements=None  LoadType=constant PQ
  A67 : PMIOPort  Tag=PMCPort  Side=Right
  B67 : PMIOPort  Tag=PMCPort  Port=2  Side=Right
  C67 : PMIOPort  Tag=PMCPort  Port=3  Side=Right
  a37 : PMIOPort  Tag=PMCPort  Port=4  Side=Right
  c37 : PMIOPort  Tag=PMCPort  Port=5  Side=Right
  b37 : PMIOPort  Tag=PMCPort  Port=6  Side=Right
  a55 : PMIOPort  Tag=PMCPort  Port=7  Side=Right
  b55 : PMIOPort  Tag=PMCPort  Port=8  Side=Right
  c55 : PMIOPort  Tag=PMCPort  Port=9  Side=Right
  A60 : PMIOPort  Tag=PMCPort  Port=10  Side=Right
  B60 : PMIOPort  Tag=PMCPort  Port=11  Side=Right
  C60 : PMIOPort  Tag=PMCPort  Port=12  Side=Right
  A37 : PMIOPort  Tag=PMCPort  Port=13  Side=Right
  B37 : PMIOPort  Tag=PMCPort  Port=14  Side=Right
  C37 : PMIOPort  Tag=PMCPort  Port=15  Side=Right
  tag scope: Pref_G2=global, Pref_G3=global
  wires:
  Pref G2/1 -> Sum4/1
  Sum5/1 -> [Pref_G3]
  Automatic Generation Control without economic dispatch process2/1(Delta_P) -> Sum4/2, Sum5/2
  Sum4/1 -> [Pref_G2]
  Pref G3/1 -> Sum5/1
  [G3_Goto] -> Automatic Generation Control without economic dispatch process2/1(dw)
  AGC ON/OFF2/1 -> Transport Delay2/1
  Transport Delay2/1 -> Automatic Generation Control without economic dispatch process2/2(AGC Status)
  connections:
  G3/LConn2 -- 03/RConn2
  62/RConn3 -- T03-62/RConn3
  T03-62/LConn1 -- 03/LConn1 -- Snubber 8/LConn1
  T03-62/LConn2 -- 03/LConn2 -- Snubber 8/LConn2
  62/RConn2 -- T03-62/RConn2
  62/RConn1 -- T03-62/RConn1
  G3/LConn3 -- 03/RConn3
  G3/LConn1 -- Load Flow Bus1/LConn1 -- 03/RConn1
  T03-62/LConn3 -- Snubber 8/LConn3 -- 03/LConn3
  78-1/RConn1 -- Load Flow Bus10/LConn1 -- 77-1/RConn1 -- 62/LConn1
  78-1/RConn2 -- 77-1/RConn2 -- 62/LConn2
  78-1/RConn3 -- 77-1/RConn3 -- 62/LConn3
  65/RConn1 -- 78-1/LConn1
  65/RConn2 -- 78-1/LConn2
  65/RConn3 -- 78-1/LConn3
  77-1/LConn1 -- 63/RConn1
  77-1/LConn2 -- 63/RConn2
  77-1/LConn3 -- 63/RConn3
  T63-64/LConn1 -- Load Flow Bus11/LConn1 -- 63/LConn1 -- 74-1/RConn1
  63/LConn2 -- T63-64/LConn2 -- 74-1/RConn2
  63/LConn3 -- T63-64/LConn3 -- 74-1/RConn3
  64/RConn1 -- T63-64/RConn1 -- T65-64/RConn1
  T63-64/RConn2 -- 64/RConn2 -- T65-64/RConn2
  T63-64/RConn3 -- 64/RConn3 -- T65-64/RConn3
  T65-64/LConn1 -- Load Flow Bus13/LConn1 -- 65/LConn1 -- 81-1/RConn1
  T65-64/LConn2 -- 81-1/RConn2 -- 65/LConn2
  T65-64/LConn3 -- 81-1/RConn3 -- 65/LConn3
  load64/LConn1 -- Load Flow Bus12/LConn1 -- 64/LConn1
  load64/LConn2 -- 64/LConn2
  load64/LConn3 -- 64/LConn3
  81-1/LConn1 -- 66/RConn1
  81-1/LConn2 -- 66/RConn2
  81-1/LConn3 -- 66/RConn3
  81-2/RConn1 -- Load Flow Bus14/LConn1 -- 66/LConn1 -- 70-1/RConn1
  81-2/RConn2 -- 66/LConn2 -- 70-1/RConn2
  81-2/RConn3 -- 66/LConn3 -- 70-1/RConn3
  81-2/LConn1 -- 67/RConn1 -- A67/RConn1
  67/RConn2 -- 81-2/LConn2 -- B67/RConn1
  C67/RConn1 -- 67/RConn3 -- 81-2/LConn3
  G2/LConn1 -- 02/RConn1
  G2/LConn2 -- 02/RConn2
  G2/LConn3 -- 02/RConn3
  02/LConn1 -- Snubber 9/LConn1 -- Load Flow Bus/LConn1 -- T02-58/LConn1
  T02-58/LConn2 -- 02/LConn2 -- Snubber 9/LConn2
  T02-58/LConn3 -- Snubber 9/LConn3 -- 02/LConn3
  T02-58/RConn1 -- 58/RConn1 -- 74-1/LConn1
  T02-58/RConn2 -- 58/RConn2 -- 74-1/LConn2
  T02-58/RConn3 -- 58/RConn3 -- 74-1/LConn3
  73-1/RConn1 -- 71-1/RConn1 -- Load Flow Bus7/LConn1 -- 58/LConn1
  71-1/RConn2 -- 73-1/RConn2 -- 58/LConn2
  71-1/RConn3 -- 73-1/RConn3 -- 58/LConn3
  71-1/LConn1 -- 57/RConn1
  71-1/LConn2 -- 57/RConn2
  71-1/LConn3 -- 57/RConn3
  73-1/LConn1 -- 59/RConn1
  73-1/LConn2 -- 59/RConn2
  73-1/LConn3 -- 59/RConn3
  75-1/RConn1 -- load59/LConn1 -- Load Flow Bus8/LConn1 -- 59/LConn1
  75-1/RConn2 -- load59/LConn2 -- 59/LConn2
  75-1/RConn3 -- load59/LConn3 -- 59/LConn3
  75-1/LConn1 -- 60/RConn1 -- 72-1/LConn1
  75-1/LConn2 -- 60/RConn2 -- 72-1/LConn2
  75-1/LConn3 -- 60/RConn3 -- 72-1/LConn3
  A60/RConn1 -- load60/LConn1 -- Load Flow Bus9/LConn1 -- 60/LConn1
  load60/LConn2 -- 60/LConn2 -- B60/RConn1
  load60/LConn3 -- C60/RConn1 -- 60/LConn3
  69-1/RConn1 -- 57/LConn1 -- 72-1/RConn1 -- Load Flow Bus6/LConn1
  57/LConn2 -- 69-1/RConn2 -- 72-1/RConn2
  57/LConn3 -- 69-1/RConn3 -- 72-1/RConn3
  69-1/LConn1 -- 56/RConn1 -- 70-1/LConn1
  69-1/LConn2 -- 56/RConn2 -- 70-1/LConn2
  56/RConn3 -- 70-1/LConn3 -- 69-1/LConn3
  68-1/RConn1 -- Load Flow Bus4/LConn1 -- load56/LConn1 -- 56/LConn1
  68-1/RConn2 -- load56/LConn2 -- 56/LConn2
  68-1/RConn3 -- load56/LConn3 -- 56/LConn3
  68-1/LConn1 -- 55/RConn1 -- 65-1/LConn1 -- a55/RConn1
  b55/RConn1 -- 55/RConn2 -- 65-1/LConn2 -- 68-1/LConn2
  65-1/LConn3 -- 68-1/LConn3 -- 55/RConn3 -- c55/RConn1
  load67/LConn1 -- Load Flow Bus15/LConn1 -- 67/LConn1
  load67/LConn2 -- 67/LConn2
  load67/LConn3 -- 67/LConn3
  65-1/RConn1 -- 52/LConn1 -- Load Flow Bus2/LConn1 -- load52/LConn1
  65-1/RConn2 -- load52/LConn2 -- 52/LConn2
  65-1/RConn3 -- load52/LConn3 -- 52/LConn3
  Load Flow Bus3/LConn1 -- 55/LConn1 -- load55/LConn1
  a37/RConn1 -- 37/RConn1
  37/RConn2 -- b37/RConn1
  37/RConn3 -- c37/RConn1
  37/LConn1 -- Load Flow Bus5/LConn1 -- 50-1/RConn1 -- A37/RConn1
  50-1/RConn2 -- B37/RConn1 -- 37/LConn2
  37/LConn3 -- 50-1/RConn3 -- C37/RConn1
  50-1/LConn1 -- 52/RConn1
  50-1/LConn2 -- 52/RConn2
  50-1/LConn3 -- 52/RConn3
  load55/LConn2 -- 55/LConn2
  load55/LConn3 -- 55/LConn3
